simulink model "greenhouse_sim"  (R2025a)
settings: Solver=ode15s  StartTime=0.0  StopTime=86400  RelTol=1e-3
settings Model: Creator=Adithiya Kumaran R K  LastModifiedBy=Adithiya Kumaran R K

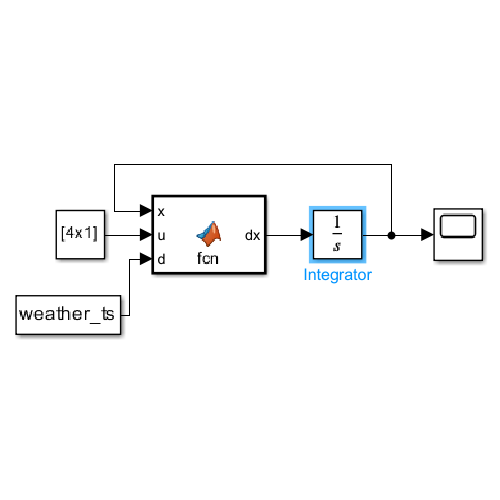
[thumbnail: Simulink's stored preview of the top-level diagram]
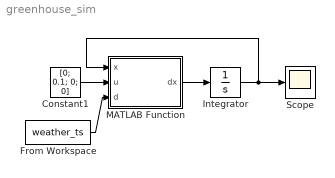
== system greenhouse_sim ==
  Constant1 : Constant  Value=[0; 0.1; 0; 0]
  From Workspace : FromWorkspace  VariableName=weather_ts
  Integrator : Integrator  InitialCondition=[15; 0.01; 400; 15; 0; 0.1; 0; 0]
  MATLAB Function : MATLAB Function  TreatAsAtomicUnit=on
  Scope : Scope
  wires:
  MATLAB Function/1(dx) -> Integrator/1
  Integrator/1 -> Scope/1, MATLAB Function/1(x)
  Constant1/1 -> MATLAB Function/2(u)
  From Workspace/1 -> MATLAB Function/3(d)

== matlab function greenhouse_sim/MATLAB Function ==
  data: x input; u input; dx output; d input
function dx = fcn(x, u, d)
    dx = greenhouse_ode(0, x, u, d);
end
